simulink model "Aerial_load_adaptive_mass"  (R2024a)
settings: Solver=FixedStepAuto  StartTime=0.0  StopTime=50  FixedStep=0.01  MaxStep=0.0001  MinStep=0.00001  RelTol=1e-9
undefined symbols (not defined in the file): F, Light, MIL
libraries: aerolibwind2 x1
settings Model: Creator=salor  LastModifiedBy=aarl0
settings SolverCC: AlgebraicLoopSolver=TrustRegion
settings DataIOCC: ReturnWorkspaceOutputs=off
settings DebuggingCC: UnconnectedInputMsg=warning  UnconnectedOutputMsg=warning  UnconnectedLineMsg=warning  ArithmeticOperatorsInVariantConditions=warning
settings ModelReferenceCC: EnableRefExpFcnMdlSchedulingChecks=on
settings SFSimCC: SimUseLocalCustomCode=off  CustomCodeUndefinedFunction=UseInterfaceOnly
settings RTWCC: RTWUseLocalCustomCode=off  GPUComputeCapability=3.5
settings CodeAppCC: StateflowObjectComments=on

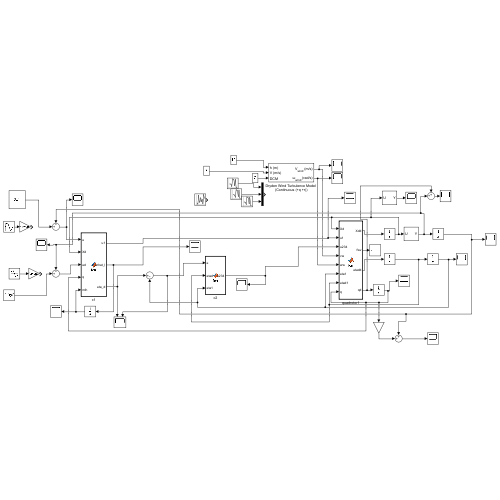
[thumbnail: Simulink's stored preview of the top-level diagram]
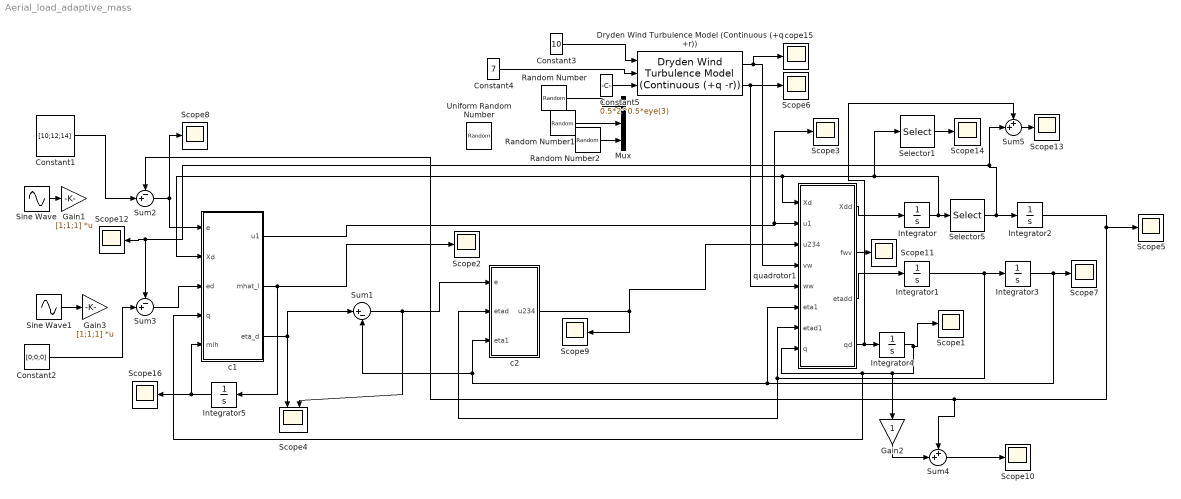
== system Aerial_load_adaptive_mass ==
  Constant1 : Constant  Value=[10;12;14]
  Constant2 : Constant  Value=[0;0;0]
  Constant3 : Constant  Value=10
  Constant4 : Constant  Value=7
  Constant5 : Constant  Value=0.5*2^0.5*eye(3)
  Dryden Wind Turbulence Model (Continuous (+q +r)) : aerolibwind2/Dryden Wind Turbulence Model  (Continuous (+q -r))  units=Metric (MKS)  spec=MIL-F-8785C  model=Continuous Dryden (+q +r)  W20=10  Wdeg=0  TurbProb=10^-2 - Light  L_high=533.4  Wingspan=10  ts=0.1  Seed=[23341 23342 23343 23344]  T_on=on
  Gain1 : Gain  Gain=[1;1;1]  Multiplication=Matrix(K*u) (u vector)
  Gain2 : Gain
  Gain3 : Gain  Gain=[1;1;1]  Multiplication=Matrix(K*u) (u vector)
  Integrator : Integrator  InitialCondition=[0;0;0;0;0;0]
  Integrator1 : Integrator  InitialCondition=[0;0;0]
  Integrator2 : Integrator  InitialCondition=[0;1;2]
  Integrator3 : Integrator  InitialCondition=[pi/60;pi/40;pi/60]
  Integrator4 : Integrator  InitialCondition=[0;0;1]
  Integrator5 : Integrator  InitialCondition=0.1
  Mux : Mux  Inputs=3
  Random Number : RandomNumber  Mean=.5  SampleTime=0.15
  Random Number1 : RandomNumber  Mean=.3  Variance=.6  Seed=0.01  SampleTime=.17
  Random Number2 : RandomNumber  Mean=.1  Variance=.25  SampleTime=.2
  Scope{1..3,5..16} (15 alike) : Scope
  Scope4 : Scope  NumInputPorts=2
  Selector1 : Selector  InputPortWidth=6  IndexOptions=Index vector (dialog)  Indices=[4:6]  OutputSizes=1
  Selector5 : Selector  InputPortWidth=6  IndexOptions=Index vector (dialog)  Indices=[1:3]  OutputSizes=1
  Sine Wave : Sin  Amplitude=0.1  Bias=10  Frequency=.4*pi  SampleTime=0
  Sine Wave1 : Sin  Amplitude=pi*0.04  Frequency=.4*pi  Phase=pi/2  SampleTime=0
  Sum1 : Sum  Inputs=|+-
  Sum2 : Sum  Inputs=-+|
  Sum3 : Sum  Inputs=-+|
  Sum4 : Sum  Inputs=++|
  Sum5 : Sum  Inputs=++|
  Uniform Random Number : UniformRandomNumber  Minimum=0.2  SampleTime=0.1
  c1 : MATLAB Function  TreatAsAtomicUnit=on
  c2 : MATLAB Function  TreatAsAtomicUnit=on
  quadrotor1 : MATLAB Function  TreatAsAtomicUnit=on
  wires:
  Integrator3/1 -> quadrotor1/6(eta1), Sum1/2, c2/3(eta1), Scope7/1
  quadrotor1/3(etadd) -> Integrator1/1
  quadrotor1/1(Xdd) -> Integrator/1
  Integrator1/1 -> quadrotor1/7(etad1), c2/2(etad), Integrator3/1
  Sum2/1 -> Scope8/1, c1/1(e)
  Sum3/1 -> c1/3(ed)
  Sine Wave/1 -> Gain1/1
  Sine Wave1/1 -> Gain3/1
  Integrator2/1 -> Sum4/1, Sum2/1, Scope5/1
  Sum1/1 -> c2/1(e), Scope4/2
  c1/3(eta_d) -> Sum1/1, Scope4/1
  c1/1(u1) -> Scope3/1, quadrotor1/2(u1)
  c2/1(u234) -> quadrotor1/3(u234), Scope9/1
  quadrotor1/4(qd) -> Integrator4/1, Sum5/1
  Integrator4/1 -> Scope1/1, c1/4(q), quadrotor1/8(q), Gain2/1
  Selector5/1 -> Integrator2/1, Scope12/1, Sum3/1, Sum5/2
  Sum4/1 -> Scope10/1
  Gain2/1 -> Sum4/2
  c1/2(mhat_l) -> Integrator5/1, Scope2/1
  quadrotor1/2(fwv) -> Scope11/1
  Random Number/1 -> Mux/1
  Random Number1/1 -> Mux/2
  Random Number2/1 -> Mux/3
  Constant1/1 -> Sum2/2
  Constant2/1 -> Sum3/2
  Sum5/1 -> Scope13/1
  Selector1/1 -> Scope14/1
  Dryden Wind Turbulence Model (Continuous (+q +r))/1 -> Scope15/1, quadrotor1/4(vw)
  Dryden Wind Turbulence Model (Continuous (+q +r))/2 -> Scope6/1, quadrotor1/5(ww)
  Constant3/1 -> Dryden Wind Turbulence Model (Continuous (+q +r))/1
  Constant5/1 -> Dryden Wind Turbulence Model (Continuous (+q +r))/3
  Constant4/1 -> Dryden Wind Turbulence Model (Continuous (+q +r))/2
  Integrator5/1 -> c1/5(mlh), Scope16/1
  Integrator/1 -> Selector1/1, c1/2(Xd), quadrotor1/1(Xd), Selector5/1

== matlab function Aerial_load_adaptive_mass/c1 ==
  data: e input; Xd input; u1 output; mhat_l output; ed input; eta_d output; q input; mlh input
function [u1,mhat_l,eta_d] = fcn(e,Xd,ed,q,mlh)

g=9.81;m_q=0.775;l=1;
landa=0.1*diag([10 10 1]);M=.05* diag([20 20 2]);gam=0.005;

w=Xd(4:6);v=Xd(1:3);
S=landa*e+ed;
ar=landa*ed;
f=g*[0;0;1]-ar;

qdot=cross(w,q);
Y=q*(q'*f+l*(w'*w));
D=qdot*q'+q*qdot';
H=Y-0.5*D*S;

F=m_q*f+mlh*H-M*S-0.1*v;

mhat_l=-gam*S'*H;
% mlhd=0;

if mlh<=0 && mhat_l<0
    mhat_l=0;
elseif mlh>=2 && mhat_l>0
    mhat_l=0;
end

u1=sqrt(F'*F);
teta_d1=atan2(F(1),F(3));
fi_d1=atan2(-F(2),sqrt(F(1)^2+F(3)^2));
eta_d=[fi_d1;teta_d1;0];

end

== matlab function Aerial_load_adaptive_mass/c2 ==
  data: u234 output; e input; etad input; eta1 input
function u234  = fcn(e,etad,eta1)
 fi1=eta1(1);teta1=eta1(2);sai=eta1(3);z=4;
% % fid=etad(1);tetad=etad(2);said=etad1(3);
% g=9.81;Ix=7.5*10^-3; Iy=7.5*10^-3;
% Iz=1.3*10^-2;Jr=6.5*10^-5;b=3.13*10^-5;
% l=0.23;m=1;

% o1=real(sqrt(complex(u1/(4*b)+u3/(2*b)-u4/(4*b))));
% o2=real(s
% m=1;
K1=.50;K2=0.10;
% k=5;
% g=9.81;
% u1=-m*(-g+K1*(z-Xq3))/(cos(fi1)*cos(teta1));

e1_q1=e(1);e1_q2=e(2);e1_q3=e(3);
fid1=etad(1);tetad1=etad(2);said1=etad(3);
u2=K1*(e1_q1)-K2*fid1;
u3=K1*(e1_q2)-K2*tetad1;
u4=K1*(e1_q3)-K2*said1;
u234=[u2;u3;u4];
end

== matlab function Aerial_load_adaptive_mass/quadrotor1 ==
  data: Xd input; u1 input; Xdd output; fwv output; u234 input; vw input; ww input; eta1 input; etad1 input; etadd output; q input; qd output
function [Xdd,fwv,etadd,qd] = fcn(Xd,u1,u234,vw,ww,eta1,etad1,q)
fi=eta1(1);teta=eta1(2);sai=eta1(3);
fid=etad1(1);tetad=etad1(2);said=etad1(3);
g=9.81;Ix=7.5*10^-3; Iy=7.5*10^-3;
Iz=1.3*10^-2;Jr=6.5*10^-5;b=3.13*10^-5;
bb=0.23;mq=0.775;ml=0.5;l=01;
VmXd=vw-Xd(1:3);wmXd=ww-Xd(4:6);
u2=u234(1);u3=u234(2);u4=u234(3);
o1=(sqrt(abs(u1/(4*b)+u3/(2*b)-u4/(4*b))));
o2=(sqrt(abs(u1/(4*b)-u2/(2*b)+u4/(4*b))));
o3=(sqrt(abs(u1/(4*b)-u3/(2*b)-u4/(4*b))));
o4=(sqrt(abs(u1/(4*b)+u2/(2*b)+u4/(4*b))));
omegar=o2+o4-o1-o3; 
a1=(Iy-Iz)/Ix; a2=Jr/Ix; a3=(Iz-Ix)/Iy; a4=Jr/Iy;
a5=(Ix-Iy)/Iz; b1=bb/Ix; b2=bb/Iy; b3=bb/Iz;
w=Xd(4:6)
mt=mq+ml;qh=[0 -q(3) q(2)
             q(3) 0 -q(1)
            -q(2) q(1) 0];e3=[0;0;1];
wh=[0 -w(3) w(2)
    w(3) 0 -w(1)
    -w(2) w(1) 0];
ro=1.22;C_dA=diag([0.05;0.05;0.1]);
kp=diag([0.1 0.1 0.1]);kr=0.12;
fww=0.5*ro*C_dA*(diag(wmXd))^2*sign(wmXd);
f1=tetad*said*a1-tetad*a2*omegar+b1*u2-kr*bb*fid/Ix;
f2=fid*said*a3+fid*a4*omegar+b2*u3-kr*bb*tetad/Iy;
f3=fid*tetad*a5+b3*u4-kr*bb*said/Iz;
etadd=([f1;f2;f3]);


fwv=0.5*ro*C_dA*(diag(VmXd))^2*sign(VmXd);
C_s=cos(sai);S_s=sin(sai);C_f=cos(fi);S_f=sin(fi);
C_t=cos(teta);S_t=sin(teta);
nw=norm(w);
R= [C_s*C_t       C_s*S_t*S_f-S_s*C_f    C_s*S_t*C_f+S_s*S_f
      S_s*C_t     C_s*C_f+S_s*S_t*S_f    S_s*S_t*C_f-C_s*S_f
        -S_t            C_t*S_f                C_t*C_f]; 
M=[mt*eye(3) -ml*l*qh;
    ml*l*qh  ml*l^2*eye(3)];
T=[fwv-kp*Xd(1:3)+mt*g*e3+ml*l*nw^2*q-u1*R*e3
    ml*g*l*qh*e3];
Xdd=inv(M)*(T);
qd=wh*q;
end
